simulink model "OSWEC_Hydraulic_Crank_PTO"  (R2018b)
settings: Solver=ode4  StartTime=0  StopTime=400  FixedStep=0.01  MaxStep=0.01  RelTol=1e-3  EnableMultiTasking=on
values from neighbouring files (symbols this model uses):
  ptosim = ptoSimClass('Non-Compressible Fluid Hydraulic')    [ptoSimInputFile.m]
undefined symbols (not defined in the file or in its folder): body, constraint, pto
libraries: PTOSim_Lib x7, WECSim_Lib x5
settings Model: Creator=mlawson  LastModifiedBy=kmruehl
settings SolverCC: ZeroCrossControl=DisableAll  AlgebraicLoopSolver=LineSearch  AutoInsertRateTranBlk=on
settings DataIOCC: SaveFormat=Array  SaveOutput=off  SaveTime=off
settings OptimizationCC: LifeSpan=inf  SimCompilerOptimization=on
settings DebuggingCC: UnderspecifiedInitializationDetection=Classic  MergeDetectMultiDrivingBlocksExec=none  SolverPrmCheckMsg=warning  AllowSymbolicDim=off  StateNameClashWarn=warning  SFUnexpectedBacktrackingDiag=warning  SFNoUnconditionalDefaultTransitionDiag=warning
settings HardwareCC: ProdBitPerPointer=32  ProdBitPerSizeT=32  ProdBitPerPtrDiffT=32  ProdLargestAtomicFloat=None  ProdIntDivRoundTo=Undefined  ProdEndianess=Unspecified  ProdWordSize=32  ProdHWDeviceType=32-bit Generic
settings ModelReferenceCC: PropagateSignalLabelsOutOfModel=off
settings SFSimCC: SimUseLocalCustomCode=off
settings RTWCC: RTWUseLocalCustomCode=off
settings CodeAppCC: StateflowObjectComments=on
settings GRTTargetCC: TargetLangStandard=C89/C90 (ANSI)  GeneratePreprocessorConditionals=Disable all
settings ConfigComp: CovMetricSettings=dw  CovHtmlReporting=on  CovSaveCumulativeToWorkspaceVar=on  CovSaveSingleToWorkspaceVar=on  CovExternalEMLEnable=off  CovSFcnEnable=off
settings SimscapeCC: SimscapeNormalizeSystem=off
settings ConfigurationSet: Description=SimMechanics 2G
settings ExplorerConfigSet: InternalSimMechanicsExplorerSettings="<ExplorerConfiguration><canonicalview>default</canonicalview><TilePanel><TileInfo><Tiles Columns=\"1\" Count=\"1\" Rows=\"1\"><Column Left=\"2\" Weight=\"1\"/><Column Left=\"1335\"/><Row Top=\"2\" Weight=\"1\"/><Row Top=\"911\"/><Tile Height=\"1\" Width=\"1\" X=\"0\" Y=\"0\"/></Tiles></TileInfo><SceneInfo><SceneViewer><BGColor><R>0.60000002384185791</R><G>0.60000002384185791</G><B>0.60000002384185791</B></BGColor><Camera><Position><X>365.37645888990272</X><Y>-369.82486814446582</Y><Z>359.64809521743916</Z></Position><Center><X>-6.7351450971904585</X><Y>2.2867358426280204</Y><Z>-12.463508769654169</Z></Center><Up><X>-0.40824829046386307</X><Y>0.40824829046386307</Y><Z>0.81649658092772615</Z></Up><Left>-57.820127362122818</Left><Right>57.820127362122818</Right><Bottom>-38.308817187253304</Bottom><Top>38.308817187253304</Top></Camera></SceneViewer></SceneInfo></TilePanel></ExplorerConfiguration>"

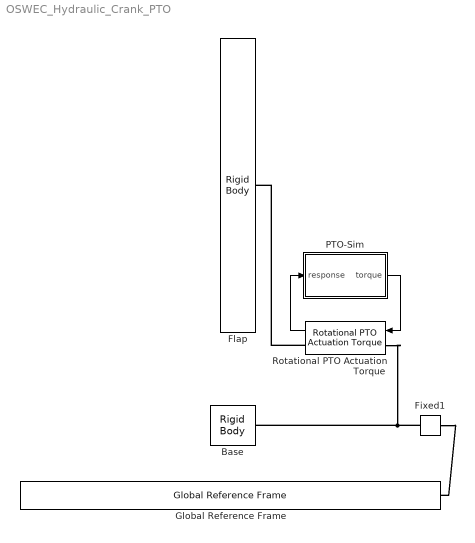
== system OSWEC_Hydraulic_Crank_PTO ==
  Base : WECSim_Lib/Body Elements/Rigid Body  body=body(2)
      settings: AttributesFormatString=%<body>  SourceProductName=WEC-Sim
  Fixed1 : WECSim_Lib/Constraints/Fixed  constraint=constraint(1)
      settings: AttributesFormatString=%<constraint>  SourceProductName=WEC-Sim
  Flap : WECSim_Lib/Body Elements/Rigid Body  body=body(1)
      settings: AttributesFormatString=%<body>  SourceProductName=WEC-Sim
  Global Reference Frame : WECSim_Lib/Frames/Global Reference Frame  waves=waves  simu=simu
      settings: SourceProductName=WEC-Sim
  PTO-Sim : Subsystem
  Rotational PTO Actuation Torque : WECSim_Lib/PTOs/Rotational PTO Actuation Torque  pto=pto(1)
      settings: AttributesFormatString=%<pto>  SourceProductName=WEC-Sim
  wires:
  Rotational PTO Actuation Torque/1 -> PTO-Sim/1(response)
  PTO-Sim/1(torque) -> Rotational PTO Actuation Torque/1
  connections:
  Fixed1/LConn1 -- Global Reference Frame/RConn1
  Fixed1/RConn1 -- Rotational PTO Actuation Torque/LConn1 -- Base/RConn1
  Rotational PTO Actuation Torque/RConn1 -- Flap/RConn1

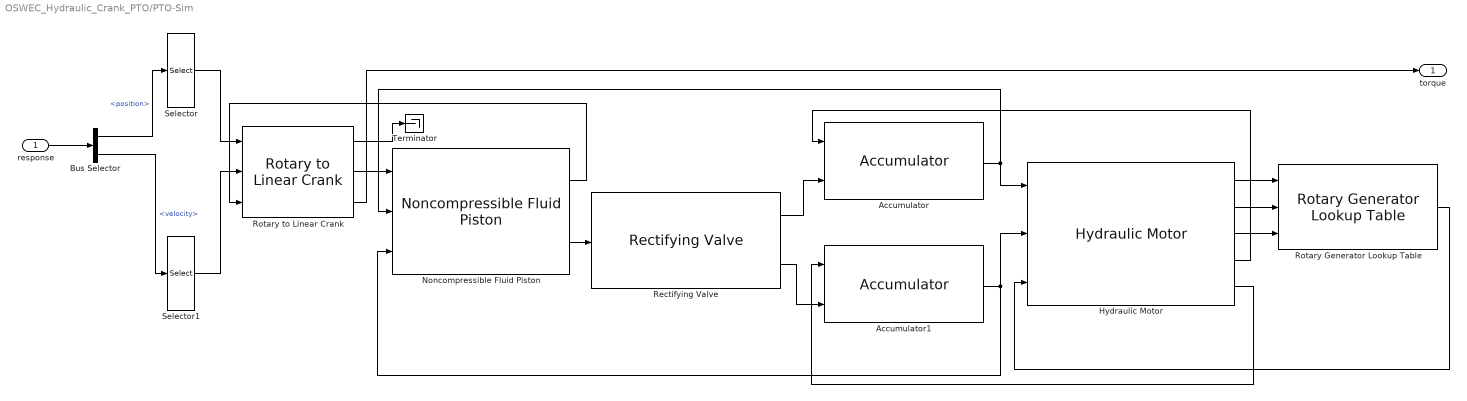
== system OSWEC_Hydraulic_Crank_PTO/PTO-Sim ==
  response : Inport
  Accumulator : PTOSim_Lib/Hydraulic/Accumulator  ptosim=ptosim.accumulator(1)
      settings: SourceProductName=PTO-Sim
  Accumulator1 : PTOSim_Lib/Hydraulic/Accumulator  ptosim=ptosim.accumulator(2)
      settings: SourceProductName=PTO-Sim
  Bus Selector : BusSelector  OutputSignals=position,velocity
  "Hydraulic Motor " : PTOSim_Lib/Hydraulic/Hydraulic Motor   ptosim=ptosim.hydraulicMotor(1)
      settings: SourceProductName=PTO-Sim
  Noncompressible Fluid Piston : PTOSim_Lib/Hydraulic/Noncompressible Fluid Piston  ptosim=ptosim.pistonNCF(1)
      settings: SourceProductName=PTO-Sim
  Rectifying Valve : PTOSim_Lib/Hydraulic/Rectifying Valve  Parameter1=ptosim.valve(1)
      settings: SourceProductName=PTO-Sim
  Rotary Generator Lookup Table : PTOSim_Lib/Generator/Rotary Generator Lookup Table  ptosim=ptosim.rotaryGenerator(1)
      settings: SourceProductName=PTO-Sim
  Rotary to Linear Crank : PTOSim_Lib/Motion Conversion/Rotary to Linear Crank  ptosim=ptosim.motionMechanism(1)
      settings: SourceProductName=PTO-Sim
  Selector : Selector  InputPortWidth=6  IndexOptions=Index vector (dialog)  Indices=5  OutputSizes=1
  Selector1 : Selector  InputPortWidth=6  IndexOptions=Index vector (dialog)  Indices=5  OutputSizes=1
  Terminator : Terminator
  torque : Outport
  wires:
  response/1 -> Bus Selector/1
  Bus Selector/1 -> Selector/1  "<position>"
  Bus Selector/2 -> Selector1/1  "<velocity>"
  Rotary to Linear Crank/3 -> torque/1
  Selector/1 -> Rotary to Linear Crank/1
  Selector1/1 -> Rotary to Linear Crank/2
  Rotary to Linear Crank/2 -> Noncompressible Fluid Piston/1
  Noncompressible Fluid Piston/2 -> Rectifying Valve/1
  Rectifying Valve/1 -> Accumulator/2
  Rectifying Valve/2 -> Accumulator1/2
  Noncompressible Fluid Piston/1 -> Rotary to Linear Crank/3
  Accumulator/1 -> "Hydraulic Motor "/1, Noncompressible Fluid Piston/2
  Accumulator1/1 -> "Hydraulic Motor "/2, Noncompressible Fluid Piston/3
  Rotary to Linear Crank/1 -> Terminator/1
  Rotary Generator Lookup Table/1 -> "Hydraulic Motor "/3
  "Hydraulic Motor "/1 -> Rotary Generator Lookup Table/1
  "Hydraulic Motor "/2 -> Rotary Generator Lookup Table/2
  "Hydraulic Motor "/3 -> Rotary Generator Lookup Table/3
  "Hydraulic Motor "/4 -> Accumulator/1
  "Hydraulic Motor "/5 -> Accumulator1/1
